simulink library "casper_library_accumulators"  (Simulink 7.2)
settings: Solver=ode45  SolverMode=SingleTasking  StartTime=0.0  StopTime=10.0  RelTol=1e-3
values from neighbouring files (symbols this model uses):
  blockCountBits = ceil(log2(numBlocks))    [address_gen_vacc_v2_mask.m]
  blockRowBits = 0    [address_gen_vacc_v2_mask.m]
  comp = compi    [bus_accumulator_init.m]    (also in bus_addsub_init.m = comp*2; bus_convert_init.m; bus_logical_init.m = comp*2; bus_maddsub_init.m = max([compa, compb, compc]))
libraries: xbsIndex_r4 x698, xbsReplacements_r4 x61, casper_library_misc x17, xps_library x9
(part 2 of 5)

== system casper_library_accumulators/simple_bram_vacc ==
  new_acc : Inport
  din : Inport  Port=2
  Adder : xbsIndex_r4/AddSub  mode=Addition  use_carryin=off  use_carryout=off  en=off  latency=2  precision=User Defined  arith_type="Signed  (2's comp)"  n_bits=n_bits  bin_pt=bin_pt  quantization=Truncate  overflow=Wrap  dbl_ovrd=off  use_behavioral_HDL=on  hw_selection=Fabric  pipelined=off  use_rpm=on  block_type=addsub
      settings: xl_area=[0, 0, 0, 0, 0, 0, 0]  block_version=10.1.3
  Constant : xbsIndex_r4/Constant  const=0  gui_display_data_type=Fixed-point  arith_type=Signed (2's comp)  n_bits=n_bits  bin_pt=bin_pt  preci_type=Single  exp_width=8  frac_width=24  explicit_period=on  period=1  equ=P=C  opselect=C  inp2=PCIN>>17  opr=+  inp1=P  carry=CIN  dbl_ovrd=off  block_type=constant
  Mux : xbsIndex_r4/Mux  inputs=2  en=off  latency=0  precision=Full  arith_type="Signed  (2's comp)"  n_bits=8  bin_pt=2  quantization=Truncate  overflow=Wrap  dbl_ovrd=off  block_type=mux
      settings: xl_area=[0, 0, 0, 0, 0, 0, 0]
  delay_bram : Subsystem  mask(delay_bram){DelayLen=vec_len - 2, bram_latency=2}
      mask prompts: DelayLen "Delay By:"; bram_latency "BRAM Latency"
      mask help: A delay block that uses BRAM for its storage.
      mask init:
      | if (DelayLen <= bram_latency)
      | 	error('delay value must be greater than BRAM Latency');
      | end
      | BitWidth = max(ceil(log2(DelayLen)), 2);
      mask Help: eval('xlWeb(''http://casper.berkeley.edu/wiki/Delay_bram'')')
  pulse_ext : Subsystem  mask(pulse_ext){pulse_len=vec_len}
      mask prompts: pulse_len "Length of Pulse"
      mask help:
      | Extends a boolean signal to be high for the specified number of clocks after
      | the last high input.
      mask init:
      | bits = ceil(log2(pulse_len+1));
      mask Help: eval('xlWeb(''http://casper.berkeley.edu/wiki/Pulse_ext'')')
  dout : Outport
  valid : Outport  Port=2
  wires:
  Constant/1 -> Mux/3
  Mux/1 -> Adder/2
  pulse_ext/1(out) -> Mux/1, valid/1
  din/1 -> Adder/1
  new_acc/1 -> pulse_ext/1(in)
  delay_bram/1(Out1) -> Mux/2, dout/1
  Adder/1 -> delay_bram/1(In1)

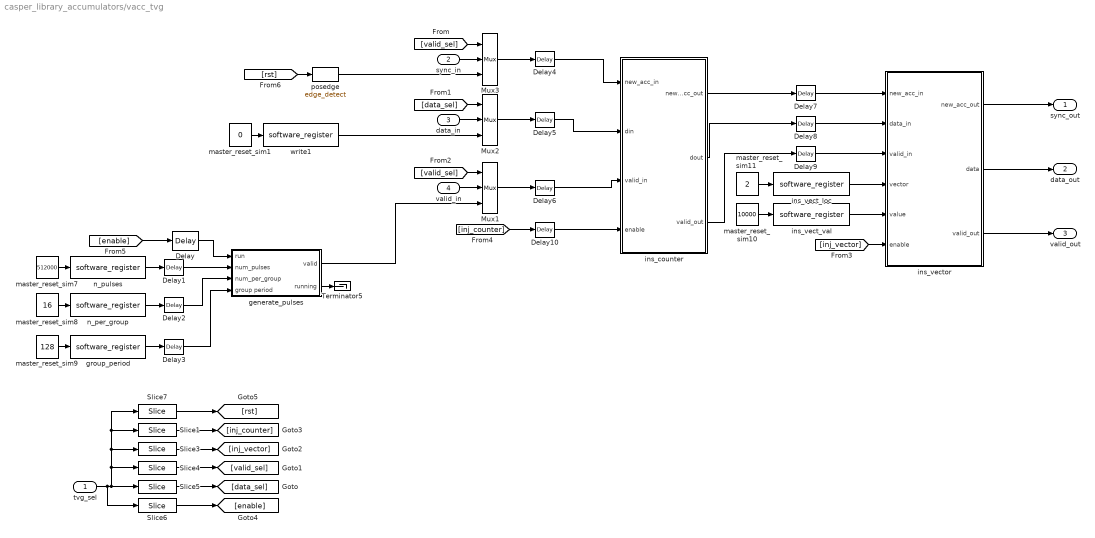
== system casper_library_accumulators/vacc_tvg ==
  tvg_sel : Inport
  sync_in : Inport  Port=2
  data_in : Inport  Port=3
  valid_in : Inport  Port=4
  Delay : xbsIndex_r4/Delay  rst=off  infoeditControl=Selection of Reset will increase slice count due to use of real FFs and instead of SRLs  en=off  latency=1  dbl_ovrd=off  reg_retiming=on  block_type=delay
      settings: xl_area=[0, 0, 0, 0, 0, 0, 0]
  Delay{1..10} (10 alike) : xbsIndex_r4/Delay  rst=off  infoeditControl=Selection of Reset will increase slice count due to use of real FFs and instead of SRLs  en=off  latency=2  dbl_ovrd=off  reg_retiming=on  block_type=delay
  Mux1 : xbsIndex_r4/Mux  inputs=2  en=off  latency=0  precision=Full  arith_type="Signed  (2's comp)"  n_bits=8  bin_pt=2  quantization=Truncate  overflow=Wrap  dbl_ovrd=off  block_type=mux
      settings: xl_area=[0, 0, 0, 0, 0, 0, 0]
  Mux2 : xbsIndex_r4/Mux  inputs=2  en=off  latency=0  precision=Full  arith_type="Signed  (2's comp)"  n_bits=8  bin_pt=2  quantization=Truncate  overflow=Wrap  dbl_ovrd=off  block_type=mux
      settings: xl_area=[0, 0, 0, 0, 0, 0, 0]
  Mux3 : xbsIndex_r4/Mux  inputs=2  en=off  latency=0  precision=Full  arith_type="Signed  (2's comp)"  n_bits=8  bin_pt=2  quantization=Truncate  overflow=Wrap  dbl_ovrd=off  block_type=mux
      settings: xl_area=[0, 0, 0, 0, 0, 0, 0]
  Slice1 : xbsIndex_r4/Slice  nbits=1  boolean_output=on  mode=Lower Bit Location + Width  bit1=0  base1=MSB of Input  bit0=4  base0=LSB of Input  dbl_ovrd=off  block_type=slice
      settings: infoedit="Extracts a given range of bits from each input sample and presents it at the output.  The output type is ordinarily unsigned with binary point at zero, but can be Boolean when the slice is one bit wide.<P><P>Hardware notes: In hardware this block costs nothing."  block_version=10.1.3
  Slice3 : xbsIndex_r4/Slice  nbits=1  boolean_output=on  mode=Lower Bit Location + Width  bit1=0  base1=MSB of Input  bit0=3  base0=LSB of Input  dbl_ovrd=off  block_type=slice
      settings: infoedit="Extracts a given range of bits from each input sample and presents it at the output.  The output type is ordinarily unsigned with binary point at zero, but can be Boolean when the slice is one bit wide.<P><P>Hardware notes: In hardware this block costs nothing."  block_version=10.1.3
  Slice4 : xbsIndex_r4/Slice  nbits=1  boolean_output=on  mode=Lower Bit Location + Width  bit1=0  base1=MSB of Input  bit0=2  base0=LSB of Input  dbl_ovrd=off  block_type=slice
      settings: infoedit="Extracts a given range of bits from each input sample and presents it at the output.  The output type is ordinarily unsigned with binary point at zero, but can be Boolean when the slice is one bit wide.<P><P>Hardware notes: In hardware this block costs nothing."  block_version=10.1.3
  Slice5 : xbsIndex_r4/Slice  nbits=1  boolean_output=on  mode=Lower Bit Location + Width  bit1=0  base1=MSB of Input  bit0=1  base0=LSB of Input  dbl_ovrd=off  block_type=slice
      settings: infoedit="Extracts a given range of bits from each input sample and presents it at the output.  The output type is ordinarily unsigned with binary point at zero, but can be Boolean when the slice is one bit wide.<P><P>Hardware notes: In hardware this block costs nothing."  block_version=10.1.3
  Slice6 : xbsIndex_r4/Slice  nbits=1  boolean_output=on  mode=Lower Bit Location + Width  bit1=0  base1=MSB of Input  bit0=0  base0=LSB of Input  dbl_ovrd=off  block_type=slice
      settings: infoedit="Extracts a given range of bits from each input sample and presents it at the output.  The output type is ordinarily unsigned with binary point at zero, but can be Boolean when the slice is one bit wide.<P><P>Hardware notes: In hardware this block costs nothing."  block_version=10.1.3
  Slice7 : xbsIndex_r4/Slice  nbits=1  boolean_output=on  mode=Lower Bit Location + Width  bit1=0  base1=MSB of Input  bit0=5  base0=LSB of Input  dbl_ovrd=off  block_type=slice
      settings: infoedit="Extracts a given range of bits from each input sample and presents it at the output.  The output type is ordinarily unsigned with binary point at zero, but can be Boolean when the slice is one bit wide.<P><P>Hardware notes: In hardware this block costs nothing."  block_version=10.1.3
  Terminator5 : Terminator
  generate_pulses : Subsystem
  group_period : xps_library/software_register  Tag=xps:sw_reg  SystemSampleTime=-1  io_dir=From Processor  arith_type=Unsigned  bitwidth=32  bin_pt=0  sample_period=1  gw_name=casper_library_accumulators_vacc_tvg_group_period_user_data_out
  ins_counter : Subsystem  mask{vec_len=len}
      mask prompts: vec_len "Vector Length?"
      mask init:
      | fmtstr = sprintf('Vector Length: %d', vec_len);
      | set_param(gcb, 'AttributesFormatString', fmtstr);
      settings: AttributesFormatString=Vector Length: 139264
  ins_vect_loc : xps_library/software_register  Tag=xps:sw_reg  SystemSampleTime=-1  io_dir=From Processor  arith_type=Unsigned  bitwidth=32  bin_pt=0  sample_period=1  gw_name=casper_library_accumulators_vacc_tvg_ins_vect_loc_user_data_out
  ins_vect_val : xps_library/software_register  Tag=xps:sw_reg  SystemSampleTime=-1  io_dir=From Processor  arith_type=Unsigned  bitwidth=32  bin_pt=0  sample_period=1  gw_name=casper_library_accumulators_vacc_tvg_ins_vect_val_user_data_out
  ins_vector : Subsystem  mask{num_vectors=len}
      mask prompts: num_vectors "number of vectors"
      mask init:
      | fmtstr = sprintf('Vector Length: %d', num_vectors);
      | set_param(gcb, 'AttributesFormatString', fmtstr);
      settings: AttributesFormatString=Vector Length: 139264
  master_reset_sim1 : Constant  Value=0
  master_reset_sim10 : Constant  Value=10000
  master_reset_sim11 : Constant  Value=2
  master_reset_sim7 : Constant  Value=512000
  master_reset_sim8 : Constant  Value=16
  master_reset_sim9 : Constant  Value=128
  n_per_group : xps_library/software_register  Tag=xps:sw_reg  SystemSampleTime=-1  io_dir=From Processor  arith_type=Unsigned  bitwidth=32  bin_pt=0  sample_period=1  gw_name=casper_library_accumulators_vacc_tvg_n_per_group_user_data_out
  n_pulses : xps_library/software_register  Tag=xps:sw_reg  SystemSampleTime=-1  io_dir=From Processor  arith_type=Unsigned  bitwidth=32  bin_pt=0  sample_period=1  gw_name=casper_library_accumulators_vacc_tvg_n_pulses_user_data_out
  posedge : casper_library_misc/edge_detect  SystemSampleTime=-1  edge=Rising  polarity=Active High  x_in=[0 0.08 0.08 0.16 0.16 0.24 0.24 0.32 0.32 0.4]  y_in="[-1 -1  1  1  1  1  1  1  1  1]"  x_out=[0.6 0.68 0.68 0.76 0.76 0.84 0.84 0.92 0.92 1]  y_out="[-1 -1  1  1 -1 -1 -1 -1 -1 -1]"
  write1 : xps_library/software_register  Tag=xps:sw_reg  SystemSampleTime=-1  io_dir=From Processor  arith_type=Unsigned  bitwidth=32  bin_pt=0  sample_period=1  gw_name=casper_library_accumulators_vacc_tvg_write1_user_data_out
  sync_out : Outport
  data_out : Outport  Port=2
  valid_out : Outport  Port=3
  wires:
  Delay10/1 -> ins_counter/4(enable)
  Delay9/1 -> ins_vector/3(valid_in)
  Delay8/1 -> ins_vector/2(data_in)
  Delay7/1 -> ins_vector/1(new_acc_in)
  Delay6/1 -> ins_counter/3(valid_in)
  Delay5/1 -> ins_counter/2(din)
  Delay4/1 -> ins_counter/1(new_acc_in)
  Delay3/1 -> generate_pulses/4(group period)
  Delay2/1 -> generate_pulses/3(num_per_group)
  Delay1/1 -> generate_pulses/2(num_pulses)
  write1/1 -> Mux2/3
  master_reset_sim1/1 -> write1/1
  [rst] -> posedge/1
  n_pulses/1 -> Delay1/1
  master_reset_sim7/1 -> n_pulses/1
  n_per_group/1 -> Delay2/1
  master_reset_sim8/1 -> n_per_group/1
  group_period/1 -> Delay3/1
  master_reset_sim9/1 -> group_period/1
  Mux1/1 -> Delay6/1
  valid_in/1 -> Mux1/2
  ins_vector/1(new_acc_out) -> sync_out/1
  ins_vector/2(data) -> data_out/1
  ins_vector/3(valid_out) -> valid_out/1
  ins_counter/1(new_acc_out) -> Delay7/1
  Mux2/1 -> Delay5/1
  data_in/1 -> Mux2/2
  sync_in/1 -> Mux3/2
  Mux3/1 -> Delay4/1
  Slice5/1 -> [data_sel]
  tvg_sel/1 -> Slice5/1, Slice3/1, Slice1/1, Slice7/1, Slice4/1, Slice6/1
  Slice4/1 -> [valid_sel]
  [valid_sel] -> Mux3/1
  [data_sel] -> Mux2/1
  [valid_sel] -> Mux1/1
  Slice3/1 -> [inj_vector]
  Slice1/1 -> [inj_counter]
  [enable] -> Delay/1
  ins_counter/2(dout) -> Delay8/1
  ins_counter/3(valid_out) -> Delay9/1
  generate_pulses/1(valid) -> Mux1/3
  posedge/1 -> Mux3/3
  [inj_vector] -> ins_vector/6(enable)
  master_reset_sim11/1 -> ins_vect_loc/1
  ins_vect_loc/1 -> ins_vector/4(vector)
  master_reset_sim10/1 -> ins_vect_val/1
  ins_vect_val/1 -> ins_vector/5(value)
  [inj_counter] -> Delay10/1
  Slice6/1 -> [enable]
  Slice7/1 -> [rst]
  Delay/1 -> generate_pulses/1(run)
  generate_pulses/2(running) -> Terminator5/1

== system casper_library_accumulators/wide_bram_vacc ==
  note: ALUMODE = 0 implements X+Y+Z+CIN
      | OPMODE selects X,Y,Z:
      | X is 0 (dv=0) or A:B (dv=1)
      | Y is 0 (acc=0) or C (acc=1)
      | Z is 0
      | CIN is CARRYIN (CARRYINSEL=0) (DSP48_low)
      | CIN is CARRYCASCIN (CARRYINSEL=2) (DSP48_high)
  new_acc : Inport
  din : Inport  Port=2
  dok : Inport  Port=3
  BitBasher : xbsIndex_r4/BitBasher  bitexpr=|  display_expr=off  sr_1=1  arith_type1="Signed  (2's comp)"  bin_pt1=0  sr_2=2  arith_type2="Signed  (2's comp)"  bin_pt2=0  sr_3=3  arith_type3=Unsigned  bin_pt3=0  sr_4=4  arith_type4=Unsigned  bin_pt4=0  dbl_ovrd=off  block_type=bitbasher
      | <!DOCTYPE HTML PUBLIC "-//W3C//DTD HTML 4.0//EN" "http://www.w3.org/TR/REC-html40/strict.dtd">
      | <html><head><meta name="qrichtext" content="1" /><style type="text/css">
      | p, li { white-space: pre-wrap; }
      | </style></head><body style=" font-family:'Sans'; font-size:10pt; font-weight:400; font-style:normal;">
      | <p style=" margin-top:12px; margin-bottom:12px; margin-left:0px; margin-right:0px; -qt-block-indent:0; text-indent:0px;"><span style=" font-family:'MS Shell Dlg'; font-size:8pt;">a={in[47:18]}<br />b={in[17:0]}</span></p></body></html>
  BitBasher1 : xbsIndex_r4/BitBasher  bitexpr=|  display_expr=off  sr_1=1  arith_type1=Unsigned  bin_pt1=0  sr_2=2  arith_type2=Unsigned  bin_pt2=0  sr_3=3  arith_type3=Unsigned  bin_pt3=0  sr_4=4  arith_type4=Unsigned  bin_pt4=0  dbl_ovrd=off  block_type=bitbasher
      | <!DOCTYPE HTML PUBLIC "-//W3C//DTD HTML 4.0//EN" "http://www.w3.org/TR/REC-html40/strict.dtd">
      | <html><head><meta name="qrichtext" content="1" /><style type="text/css">
      | p, li { white-space: pre-wrap; }
      | </style></head><body style=" font-family:'Sans'; font-size:10pt; font-weight:400; font-style:normal;">
      | <p style=" margin-top:12px; margin-bottom:12px; margin-left:0px; margin-right:0px; -qt-block-indent:0; text-indent:0px;"><span style=" font-family:'MS Shell Dlg'; font-size:8pt;">op={3'b000, acc, acc, dv, dv}</span></p></body></html>
  BitBasher3 : xbsIndex_r4/BitBasher  bitexpr=|  display_expr=off  sr_1=1  arith_type1="Signed  (2's comp)"  bin_pt1=0  sr_2=2  arith_type2="Signed  (2's comp)"  bin_pt2=0  sr_3=3  arith_type3=Unsigned  bin_pt3=0  sr_4=4  arith_type4=Unsigned  bin_pt4=0  dbl_ovrd=off  block_type=bitbasher
      | <!DOCTYPE HTML PUBLIC "-//W3C//DTD HTML 4.0//EN" "http://www.w3.org/TR/REC-html40/strict.dtd">
      | <html><head><meta name="qrichtext" content="1" /><style type="text/css">
      | p, li { white-space: pre-wrap; }
      | </style></head><body style=" font-family:'Sans'; font-size:10pt; font-weight:400; font-style:normal;">
      | <p style=" margin-top:12px; margin-bottom:12px; margin-left:0px; margin-right:0px; -qt-block-indent:0; text-indent:0px;"><span style=" font-family:'MS Shell Dlg'; font-size:8pt;">a={in[47:18]}<br />b={in[17:0]}</span></p></body></html>
  Constant10 : xbsIndex_r4/Constant  const=2  gui_display_data_type=Fixed-point  arith_type=Unsigned  n_bits=3  bin_pt=0  preci_type=Single  exp_width=8  frac_width=24  explicit_period=on  period=1  equ=P=C  opselect=C  inp2=PCIN>>17  opr=+  inp1=P  carry=CIN  dbl_ovrd=off  block_type=constant
  Constant11 : xbsIndex_r4/Constant  const=0  gui_display_data_type=Fixed-point  arith_type=Unsigned  n_bits=4  bin_pt=0  preci_type=Single  exp_width=8  frac_width=24  explicit_period=off  period=1  equ=P=C  opselect=C  inp2=PCIN>>17  opr=+  inp1=P  carry=CIN  dbl_ovrd=off  block_type=constant
  Constant12 : xbsIndex_r4/Constant  const=0  gui_display_data_type=Fixed-point  arith_type=Unsigned  n_bits=1  bin_pt=0  preci_type=Single  exp_width=8  frac_width=24  explicit_period=on  period=1  equ=P=C  opselect=C  inp2=PCIN>>17  opr=+  inp1=P  carry=CIN  dbl_ovrd=off  block_type=constant
  Constant13 : xbsIndex_r4/Constant  const=0  gui_display_data_type=Fixed-point  arith_type=Unsigned  n_bits=3  bin_pt=0  preci_type=Single  exp_width=8  frac_width=24  explicit_period=on  period=1  equ=P=C  opselect=C  inp2=PCIN>>17  opr=+  inp1=P  carry=CIN  dbl_ovrd=off  block_type=constant
  Constant8 : xbsIndex_r4/Constant  const=0  gui_display_data_type=Fixed-point  arith_type=Unsigned  n_bits=4  bin_pt=0  preci_type=Single  exp_width=8  frac_width=24  explicit_period=on  period=1  equ=P=C  opselect=C  inp2=PCIN>>17  opr=+  inp1=P  carry=CIN  dbl_ovrd=off  block_type=constant
  Constant9 : xbsIndex_r4/Constant  const=0  gui_display_data_type=Fixed-point  arith_type=Unsigned  n_bits=1  bin_pt=0  preci_type=Single  exp_width=8  frac_width=24  explicit_period=on  period=1  equ=P=C  opselect=C  inp2=PCIN>>17  opr=+  inp1=P  carry=CIN  dbl_ovrd=off  block_type=constant
  DSP48E1_high : xbsIndex_r4/DSP48E1   use_a=Direct from A Port  use_b=Direct from B Port  addsub_mode=ONE48  xl_useadderonly=on  xl_dynamicmult=off  enable_preadder=off  reset_preg=off  pattern_from_creg=1  pattern='000000000000'  mask_from_creg=1  pattern_mask='000000000000'  use_op=off  use_creg=on  rst_all=off  en_all=off  use_pcin=off  use_carrycascin=on  use_multsignin=off  use_carryout=off  use_patterndetect=off  use_patternbdetect=off  use_overflow=off  use_underflow=off  use_acout=off  use_bcout=off  use_pcout=off  use_multsignout=off  use_carrycascout=off  pipeline_a=2  pipeline_b=2  pipeline_acout=1  pipeline_bcout=1  pipeline_c=on  pipeline_p=on  pipeline_mult=off  pipeline_opmode=on  pipeline_alumode=off  pipeline_carryin=off  pipeline_carryinsel=off  dreg=off  adreg=off  register_inmode=off  rst_a=off  rst_b=off  rst_c=off  rst_mult=off  rst_p=off  rst_carry_in=off  rst_alumode=off  rst_ctrl=off  reset_port_d=off  reset_port_inmode=off  en_a1=off  en_a2=off  en_b1=off  en_b2=off  en_c=off  en_mult=off  en_p=off  en_carry_in=off  en_alumode=off  en_multcarryin=off  en_ctrl=off  enable_port_regd=off  enable_port_regad=off  enable_port_reginmode=off  use_synth_model=off  block_type=dsp48e1
  DSP48E1_low : xbsIndex_r4/DSP48E1   use_a=Direct from A Port  use_b=Direct from B Port  addsub_mode=ONE48  xl_useadderonly=on  xl_dynamicmult=off  enable_preadder=off  reset_preg=off  pattern_from_creg=1  pattern='000000000000'  mask_from_creg=1  pattern_mask='000000000000'  use_op=off  use_creg=on  rst_all=off  en_all=off  use_pcin=off  use_carrycascin=off  use_multsignin=off  use_carryout=off  use_patterndetect=off  use_patternbdetect=off  use_overflow=off  use_underflow=off  use_acout=off  use_bcout=off  use_pcout=off  use_multsignout=off  use_carrycascout=on  pipeline_a=1  pipeline_b=1  pipeline_acout=1  pipeline_bcout=1  pipeline_c=on  pipeline_p=on  pipeline_mult=off  pipeline_opmode=on  pipeline_alumode=off  pipeline_carryin=off  pipeline_carryinsel=off  dreg=off  adreg=off  register_inmode=off  rst_a=off  rst_b=off  rst_c=off  rst_mult=off  rst_p=off  rst_carry_in=off  rst_alumode=off  rst_ctrl=off  reset_port_d=off  reset_port_inmode=off  en_a1=off  en_a2=off  en_b1=off  en_b2=off  en_c=off  en_mult=off  en_p=off  en_carry_in=off  en_alumode=off  en_multcarryin=off  en_ctrl=off  enable_port_regd=off  enable_port_regad=off  enable_port_reginmode=off  use_synth_model=off  block_type=dsp48e1
  Delay : xbsIndex_r4/Delay  rst=off  infoeditControl=Selection of Reset will increase slice count due to use of real FFs and instead of SRLs  en=off  latency=1  dbl_ovrd=off  reg_retiming=on  block_type=delay
  Delay1 : xbsIndex_r4/Delay  rst=off  infoeditControl=Selection of Reset will increase slice count due to use of real FFs and instead of SRLs  en=off  latency=1  dbl_ovrd=off  reg_retiming=on  block_type=delay
  Delay2 : xbsIndex_r4/Delay  rst=off  infoeditControl=Selection of Reset will increase slice count due to use of real FFs and instead of SRLs  en=off  latency=1  dbl_ovrd=off  reg_retiming=on  block_type=delay
  Inverter : xbsIndex_r4/Inverter  en=off  latency=0  dbl_ovrd=off  block_type=inv
  delay_bram_high : Subsystem  mask(delay_bram){DelayLen=vec_len - 2, bram_latency=2}
      mask prompts: DelayLen "Delay By:"; bram_latency "BRAM Latency"
      mask help: A delay block that uses BRAM for its storage.
      mask init:
      | if (DelayLen <= bram_latency)
      | 	error('delay value must be greater than BRAM Latency');
      | end
      | BitWidth = max(ceil(log2(DelayLen)), 2);
      mask Help: eval('xlWeb(''http://casper.berkeley.edu/wiki/Delay_bram'')')
  delay_bram_low : Subsystem  mask(delay_bram){DelayLen=vec_len - 2, bram_latency=2}
      mask prompts: DelayLen "Delay By:"; bram_latency "BRAM Latency"
      mask help: A delay block that uses BRAM for its storage.
      mask init:
      | if (DelayLen <= bram_latency)
      | 	error('delay value must be greater than BRAM Latency');
      | end
      | BitWidth = max(ceil(log2(DelayLen)), 2);
      mask Help: eval('xlWeb(''http://casper.berkeley.edu/wiki/Delay_bram'')')
  insize : Subsystem
  outsize : Subsystem
  pulse_ext : Subsystem  mask(pulse_ext){pulse_len=vec_len}
      mask prompts: pulse_len "Length of Pulse"
      mask help:
      | Extends a boolean signal to be high for the specified number of clocks after
      | the last high input.
      mask init:
      | bits = ceil(log2(pulse_len+1));
      mask Help: eval('xlWeb(''http://casper.berkeley.edu/wiki/Pulse_ext'')')
  dout : Outport
  valid : Outport  Port=2
  wires:
  new_acc/1 -> pulse_ext/1(in)  "new_acc"
  pulse_ext/1(out) -> Inverter/1, Delay2/1  "init"
  DSP48E1_low/2 -> DSP48E1_high/8  "carry"
  BitBasher/1 -> DSP48E1_low/1  "lo_a"
  BitBasher/2 -> DSP48E1_low/2  "lo_b"
  DSP48E1_low/1 -> delay_bram_low/1(In1)  "lo_p"
  delay_bram_low/1(Out1) -> Delay/1, DSP48E1_low/3  "lo_c"
  BitBasher1/1 -> Delay1/1, DSP48E1_low/4  "lo_op"
  Inverter/1 -> BitBasher1/1  "acc"
  dok/1 -> BitBasher1/2  "dok"
  BitBasher3/1 -> DSP48E1_high/1  "hi_a"
  BitBasher3/2 -> DSP48E1_high/2  "hi_b"
  Delay1/1 -> DSP48E1_high/4  "hi_op"
  Constant8/1 -> DSP48E1_high/5
  Constant9/1 -> DSP48E1_high/6
  Constant10/1 -> DSP48E1_high/7
  DSP48E1_high/1 -> delay_bram_high/1(In1)  "hi_p"
  Constant11/1 -> DSP48E1_low/5
  Constant12/1 -> DSP48E1_low/6
  Constant13/1 -> DSP48E1_low/7
  din/1 -> insize/1(in)  "din"
  insize/2(lo) -> BitBasher/1  "lo"
  delay_bram_high/1(Out1) -> outsize/1(hi), DSP48E1_high/3  "hi_c"
  insize/1(hi) -> BitBasher3/1  "hi"
  Delay/1 -> outsize/2(lo)  "lo_c1"
  outsize/1(out) -> dout/1  "dout"
  Delay2/1 -> valid/1  "valid"

== system casper_library_accumulators/addr_bram_vacc/delay_bram ==
  In1 : Inport
  Constant2 : xbsIndex_r4/Constant  const=1  gui_display_data_type=Fixed-point  arith_type=Boolean  n_bits=1  bin_pt=0  preci_type=Single  exp_width=8  frac_width=24  explicit_period=on  period=1  equ=P=C  opselect=C  inp2=PCIN>>17  opr=+  inp1=P  carry=CIN  dbl_ovrd=off  block_type=constant
  Counter : xbsIndex_r4/Counter  cnt_type=Count Limited  cnt_to=DelayLen - bram_latency - 1  operation=Up  start_count=0  cnt_by_val=1  arith_type=Unsigned  n_bits=BitWidth  bin_pt=0  load_pin=off  rst=off  en=off  explicit_period=off  period=1  dbl_ovrd=off  use_behavioral_HDL=on  implementation=Fabric  use_rpm=off  block_type=counter
      settings: xl_area=[0, 0, 0, 0, 0, 0, 0]
  Single Port RAM : xbsIndex_r4/Single Port RAM  depth=2^BitWidth  initVector=0  distributed_mem=Block RAM  write_mode=Read Before Write  rst=off  init_reg=0  en=off  latency=bram_latency  dbl_ovrd=off  optimize=Area  use_rpm=off  block_type=spram
      settings: xl_area=[0, 0, 0, 0, 0, 0, 0]  block_version=10.1.3
  Out1 : Outport
  wires:
  Single Port RAM/1 -> Out1/1
  Counter/1 -> Single Port RAM/1
  In1/1 -> Single Port RAM/2
  Constant2/1 -> Single Port RAM/3

== system casper_library_accumulators/addr_bram_vacc/pulse_ext ==
  in : Inport
  Constant5 : xbsIndex_r4/Constant  const=pulse_len  gui_display_data_type=Fixed-point  arith_type=Unsigned  n_bits=bits  bin_pt=0  preci_type=Single  exp_width=8  frac_width=24  explicit_period=off  period=1  equ=P=C  opselect=C  inp2=PCIN>>17  opr=+  inp1=P  carry=CIN  dbl_ovrd=off  block_type=constant
  Counter3 : xbsIndex_r4/Counter  cnt_type=Free Running  cnt_to=1023  operation=Up  start_count=0  cnt_by_val=1  arith_type=Unsigned  n_bits=bits  bin_pt=0  load_pin=off  rst=on  en=on  explicit_period=on  period=1  dbl_ovrd=off  use_behavioral_HDL=on  implementation=Fabric  use_rpm=on  block_type=counter
      settings: xl_area=[0, 0, 0, 0, 0, 0, 0]
  Relational5 : xbsIndex_r4/Relational  mode=a!=b  en=off  latency=0  dbl_ovrd=off  block_type=relational
      settings: xl_area=[0, 0, 0, 0, 0, 0, 0]  block_version=10.1.3
  posedge : Subsystem  Tag=Rising Edge Detector
  out : Outport
  wires:
  posedge/1(Out) -> Counter3/1
  in/1 -> posedge/1(In)
  Relational5/1 -> out/1, Counter3/2
  Constant5/1 -> Relational5/2
  Counter3/1 -> Relational5/1

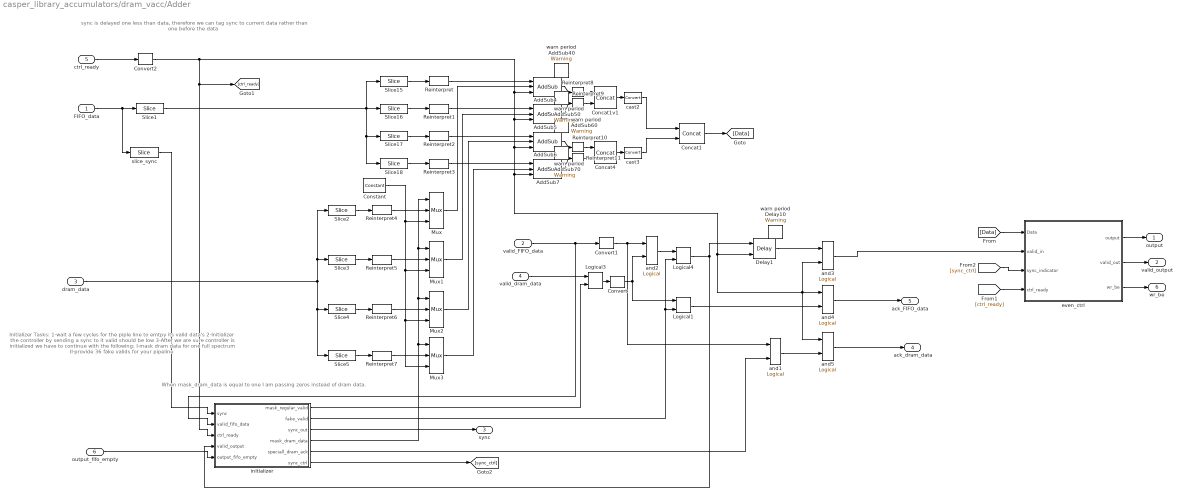
== system casper_library_accumulators/dram_vacc/Adder ==
  note: When mask_dram_data is equal to one
      | I am passing zeros instead of dram data.
  note: Initializer Tasks:
      | 1-wait a few cycles for the piple line to emtpy
      | its valid data's
      | 2-Initializer the controller by sending a sync to it
      | valid should be low
      | 3-After we are sure controller is initialized we have to
      | continue with the following:
      | I-mask dram data for one full spectrum
      | II-provide 36 fake valids for your pipeline
  note: sync is delayed one less than data,
      | therefore we can tag sync to current data rather than
      | one before the data
  FIFO_data : Inport
  valid_FIFO_data : Inport  Port=2
  dram_data : Inport  Port=3
  valid_dram_data : Inport  Port=4
  ctrl_ready : Inport  Port=5
  output_fifo_empty : Inport  Port=6
  AddSub{4..7} (4 alike) : xbsIndex_r4/AddSub  mode=Addition  use_carryin=off  use_carryout=off  en=on  latency=3  precision=User Defined  arith_type="Signed  (2's comp)"  n_bits=32  bin_pt=0  quantization="Round  (unbiased: +/- Inf)"  overflow=Wrap  dbl_ovrd=off  use_behavioral_HDL=on  hw_selection=Fabric  pipelined=on  use_rpm=on  block_type=addsub
      settings: xl_area=[0, 0, 0, 0, 0, 0, 0]  block_version=9.2.01
  Concat1 : xbsIndex_r4/Concat  num_inputs=2  dbl_ovrd=off  block_type=concat
      settings: block_version=9.2.01
  Concat1v1 : xbsIndex_r4/Concat  num_inputs=2  dbl_ovrd=off  block_type=concat
      settings: block_version=9.2.01
  Concat4 : xbsIndex_r4/Concat  num_inputs=2  dbl_ovrd=off  block_type=concat
      settings: block_version=9.2.01
  Constant : xbsIndex_r4/Constant  const=0  gui_display_data_type=Fixed-point  arith_type=Signed (2's comp)  n_bits=32  bin_pt=0  preci_type=Single  exp_width=8  frac_width=24  explicit_period=on  period=1  equ=P=C  opselect=C  inp2=PCIN>>17  opr=+  inp1=P  carry=CIN  dbl_ovrd=off  block_type=constant
      settings: block_version=9.2.01
  Convert : xbsIndex_r4/Convert  gui_display_data_type=Fixed-point  arith_type=Boolean  n_bits=8  bin_pt=6  float_type=Single  exp_bits=8  fraction_bits=24  quantization=Truncate  overflow=Wrap  en=off  latency=0  dbl_ovrd=off  pipeline=off  block_type=convert
      settings: xl_area=[0, 0, 0, 0, 0, 0, 0]  block_version=9.2.01
  Convert1 : xbsIndex_r4/Convert  gui_display_data_type=Fixed-point  arith_type=Boolean  n_bits=8  bin_pt=6  float_type=Single  exp_bits=8  fraction_bits=24  quantization=Truncate  overflow=Wrap  en=off  latency=0  dbl_ovrd=off  pipeline=off  block_type=convert
      settings: xl_area=[0, 0, 0, 0, 0, 0, 0]  block_version=9.2.01
  Convert2 : xbsIndex_r4/Convert  gui_display_data_type=Fixed-point  arith_type=Boolean  n_bits=8  bin_pt=6  float_type=Single  exp_bits=8  fraction_bits=24  quantization=Truncate  overflow=Wrap  en=off  latency=0  dbl_ovrd=off  pipeline=off  block_type=convert
      settings: xl_area=[0, 0, 0, 0, 0, 0, 0]  block_version=9.2.01
  Delay1 : xbsIndex_r4/Delay  rst=off  infoeditControl=Selection of Reset will increase slice count due to use of real FFs and instead of SRLs  en=on  latency=3  dbl_ovrd=off  reg_retiming=on  block_type=delay
      settings: xl_area=[0, 0, 0, 0, 0, 0, 0]  block_version=9.2.01
  Logical1 : xbsIndex_r4/Logical  logical_function=OR  inputs=2  en=off  latency=0  precision=Full  arith_type=Unsigned  n_bits=8  bin_pt=2  align_bp=on  dbl_ovrd=off  block_type=logical
      settings: xl_area=[0, 0, 0, 0, 0, 0, 0]  block_version=9.2.01
  Logical3 : xbsIndex_r4/Logical  logical_function=AND  inputs=2  en=off  latency=0  precision=Full  arith_type=Unsigned  n_bits=8  bin_pt=2  align_bp=on  dbl_ovrd=off  block_type=logical
      settings: xl_area=[0, 0, 0, 0, 0, 0, 0]  block_version=9.2.01
  Logical4 : xbsIndex_r4/Logical  logical_function=OR  inputs=2  en=off  latency=0  precision=Full  arith_type=Unsigned  n_bits=8  bin_pt=2  align_bp=on  dbl_ovrd=off  block_type=logical
      settings: xl_area=[0, 0, 0, 0, 0, 0, 0]  block_version=9.2.01
  Mux{,1..3} (4 alike) : xbsIndex_r4/Mux  inputs=2  en=off  latency=0  precision=Full  arith_type="Signed  (2's comp)"  n_bits=8  bin_pt=2  quantization=Truncate  overflow=Wrap  dbl_ovrd=off  block_type=mux
      settings: xl_area=[0, 0, 0, 0, 0, 0, 0]  block_version=9.2.01
  Reinterpret{,1..7} (8 alike) : xbsIndex_r4/Reinterpret  force_arith_type=on  arith_type="Signed  (2's comp)"  force_bin_pt=on  bin_pt=0  block_type=reinterpret
      settings: infoedit="Changes signal type without altering the binary representation.   You can changed the signal between signed and unsigned, and relocate the binary point.<P><P>Hardware notes: In hardware this block costs nothing.<P><P>Example:  Suppose the input is 6 bits wide, signed, with 2 fractional bits, and the output is forced to unsigned with 0 fractional bits.  Then an input of -2.0 (1110.00 in binary 2's complement) becomes an output of 56 (111000 in binary)."  block_version=9.2.01
  Reinterpret{8..11} (4 alike) : xbsIndex_r4/Reinterpret  force_arith_type=on  arith_type=Unsigned  force_bin_pt=on  bin_pt=0  block_type=reinterpret
      settings: infoedit="Changes signal type without altering the binary representation.   You can changed the signal between signed and unsigned, and relocate the binary point.<P><P>Hardware notes: In hardware this block costs nothing.<P><P>Example:  Suppose the input is 6 bits wide, signed, with 2 fractional bits, and the output is forced to unsigned with 0 fractional bits.  Then an input of -2.0 (1110.00 in binary 2's complement) becomes an output of 56 (111000 in binary)."  block_version=9.2.01
  Slice1 : xbsIndex_r4/Slice  nbits=128  boolean_output=off  mode=Lower Bit Location + Width  bit1=0  base1=MSB of Input  bit0=0  base0=LSB of Input  dbl_ovrd=off  block_type=slice
      settings: infoedit="Extracts a given range of bits from each input sample and presents it at the output.  The output type is ordinarily unsigned with binary point at zero, but can be Boolean when the slice is one bit wide.<P><P>Hardware notes: In hardware this block costs nothing."  block_version=9.2.01
  Slice15 : xbsIndex_r4/Slice  nbits=32  boolean_output=off  mode=Lower Bit Location + Width  bit1=96  base1=MSB of Input  bit0=96  base0=LSB of Input  dbl_ovrd=off  block_type=slice
      settings: infoedit="Extracts a given range of bits from each input sample and presents it at the output.  The output type is ordinarily unsigned with binary point at zero, but can be Boolean when the slice is one bit wide.<P><P>Hardware notes: In hardware this block costs nothing."  block_version=9.2.01
  Slice16 : xbsIndex_r4/Slice  nbits=32  boolean_output=off  mode=Lower Bit Location + Width  bit1=-32  base1=MSB of Input  bit0=64  base0=LSB of Input  dbl_ovrd=off  block_type=slice
      settings: infoedit="Extracts a given range of bits from each input sample and presents it at the output.  The output type is ordinarily unsigned with binary point at zero, but can be Boolean when the slice is one bit wide.<P><P>Hardware notes: In hardware this block costs nothing."  block_version=9.2.01
  Slice17 : xbsIndex_r4/Slice  nbits=32  boolean_output=off  mode=Lower Bit Location + Width  bit1=0  base1=MSB of Input  bit0=32  base0=LSB of Input  dbl_ovrd=off  block_type=slice
      settings: infoedit="Extracts a given range of bits from each input sample and presents it at the output.  The output type is ordinarily unsigned with binary point at zero, but can be Boolean when the slice is one bit wide.<P><P>Hardware notes: In hardware this block costs nothing."  block_version=9.2.01
  Slice18 : xbsIndex_r4/Slice  nbits=32  boolean_output=off  mode=Lower Bit Location + Width  bit1=0  base1=MSB of Input  bit0=0  base0=LSB of Input  dbl_ovrd=off  block_type=slice
      settings: infoedit="Extracts a given range of bits from each input sample and presents it at the output.  The output type is ordinarily unsigned with binary point at zero, but can be Boolean when the slice is one bit wide.<P><P>Hardware notes: In hardware this block costs nothing."  block_version=9.2.01
  Slice2 : xbsIndex_r4/Slice  nbits=32  boolean_output=off  mode=Lower Bit Location + Width  bit1=0  base1=MSB of Input  bit0=104  base0=LSB of Input  dbl_ovrd=off  block_type=slice
      settings: infoedit="Extracts a given range of bits from each input sample and presents it at the output.  The output type is ordinarily unsigned with binary point at zero, but can be Boolean when the slice is one bit wide.<P><P>Hardware notes: In hardware this block costs nothing."  block_version=9.2.01
  Slice3 : xbsIndex_r4/Slice  nbits=32  boolean_output=off  mode=Lower Bit Location + Width  bit1=72  base1=MSB of Input  bit0=72  base0=LSB of Input  dbl_ovrd=off  block_type=slice
      settings: infoedit="Extracts a given range of bits from each input sample and presents it at the output.  The output type is ordinarily unsigned with binary point at zero, but can be Boolean when the slice is one bit wide.<P><P>Hardware notes: In hardware this block costs nothing."  block_version=9.2.01
  Slice4 : xbsIndex_r4/Slice  nbits=32  boolean_output=off  mode=Lower Bit Location + Width  bit1=0  base1=MSB of Input  bit0=32  base0=LSB of Input  dbl_ovrd=off  block_type=slice
      settings: infoedit="Extracts a given range of bits from each input sample and presents it at the output.  The output type is ordinarily unsigned with binary point at zero, but can be Boolean when the slice is one bit wide.<P><P>Hardware notes: In hardware this block costs nothing."  block_version=9.2.01
  Slice5 : xbsIndex_r4/Slice  nbits=32  boolean_output=off  mode=Lower Bit Location + Width  bit1=0  base1=MSB of Input  bit0=0  base0=LSB of Input  dbl_ovrd=off  block_type=slice
      settings: infoedit="Extracts a given range of bits from each input sample and presents it at the output.  The output type is ordinarily unsigned with binary point at zero, but can be Boolean when the slice is one bit wide.<P><P>Hardware notes: In hardware this block costs nothing."  block_version=9.2.01
  and1 : xbsIndex_r4/Logical  logical_function=OR  inputs=2  en=off  latency=0  precision=Full  arith_type=Unsigned  n_bits=8  bin_pt=2  align_bp=on  dbl_ovrd=off  block_type=logical
      settings: xl_area=[0, 0, 0, 0, 0, 0, 0]  block_version=9.2.01
  and{2..5} (4 alike) : xbsIndex_r4/Logical  logical_function=AND  inputs=2  en=off  latency=0  precision=Full  arith_type=Unsigned  n_bits=8  bin_pt=2  align_bp=on  dbl_ovrd=off  block_type=logical
      settings: xl_area=[0, 0, 0, 0, 0, 0, 0]  block_version=9.2.01
  cast2 : xbsIndex_r4/Convert  gui_display_data_type=Fixed-point  arith_type=Unsigned  n_bits=72  bin_pt=0  float_type=Single  exp_bits=8  fraction_bits=24  quantization=Truncate  overflow=Wrap  en=off  latency=0  dbl_ovrd=off  pipeline=off  block_type=convert
      settings: xl_area=[0, 0, 0, 0, 0, 0, 0]  block_version=9.2.01
  cast3 : xbsIndex_r4/Convert  gui_display_data_type=Fixed-point  arith_type=Unsigned  n_bits=72  bin_pt=0  float_type=Single  exp_bits=8  fraction_bits=24  quantization=Truncate  overflow=Wrap  en=off  latency=0  dbl_ovrd=off  pipeline=off  block_type=convert
      settings: xl_area=[0, 0, 0, 0, 0, 0, 0]  block_version=9.2.01
  even_ctrl : Subsystem
  initializer : Subsystem
  slice_sync : xbsIndex_r4/Slice  nbits=1  boolean_output=on  mode=Upper Bit Location + Width  bit1=0  base1=MSB of Input  bit0=0  base0=LSB of Input  dbl_ovrd=off  block_type=slice
      settings: infoedit="Extracts a given range of bits from each input sample and presents it at the output.  The output type is ordinarily unsigned with binary point at zero, but can be Boolean when the slice is one bit wide.<P><P>Hardware notes: In hardware this block costs nothing."  block_version=9.2.01
  warn period AddSub{40,50,60,70} (4 alike) : xbsReplacements_r4/Warning  SystemSampleTime=-1  period=1
  warn period Delay10 : xbsReplacements_r4/Warning  SystemSampleTime=-1  period=1
  output : Outport
  valid_output : Outport  Port=2
  sync : Outport  Port=3
  ack_dram_data : Outport  Port=4
  ack_FIFO_data : Outport  Port=5
  wr_be : Outport  Port=6
  wires:
  Reinterpret11/1 -> Concat4/2
  Reinterpret10/1 -> Concat4/1
  Reinterpret9/1 -> Concat1v1/2
  Reinterpret8/1 -> Concat1v1/1
  Reinterpret7/1 -> Mux3/2
  Reinterpret6/1 -> Mux2/2
  Reinterpret5/1 -> Mux1/2
  Reinterpret4/1 -> Mux/2
  Reinterpret3/1 -> AddSub7/1
  Reinterpret2/1 -> AddSub6/1
  Reinterpret1/1 -> AddSub5/1
  Reinterpret/1 -> AddSub4/1
  Logical1/1 -> and4/2
  and1/1 -> and5/2
  and5/1 -> ack_dram_data/1
  Logical4/1 -> initializer/4(valid_output), Delay1/1
  initializer/5(speciall_dram_ack) -> and1/2
  output_fifo_empty/1 -> initializer/5(output_fifo_empty)
  Constant/1 -> Mux2/3, Mux3/3, Mux1/3, Mux/3
  initializer/4(mask_dram_data) -> Mux3/1, Mux2/1, Mux1/1, Mux/1
  Slice2/1 -> Reinterpret4/1
  Slice3/1 -> Reinterpret5/1
  Slice4/1 -> Reinterpret6/1
  Slice5/1 -> Reinterpret7/1
  initializer/3(sync_out) -> sync/1
  and2/1 -> Logical4/1
  and4/1 -> ack_FIFO_data/1
  Delay1/1 -> and3/1
  initializer/2(fake_valid) -> Logical1/2, Logical4/2
  Logical3/1 -> Convert/1
  initializer/1(mask_regular_valid) -> Logical3/2
  valid_dram_data/1 -> Logical3/1
  and3/1 -> even_ctrl/2(valid_in)
  Convert2/1 -> [ctrl_ready], initializer/3(ctrl_ready), AddSub4/3, AddSub5/3, Delay1/2, and5/1, and4/1, and3/2, AddSub7/3, AddSub6/3
  Convert1/1 -> and1/1, and2/1
  Convert/1 -> Logical1/1, and2/2
  slice_sync/1 -> initializer/1(sync)
  Slice1/1 -> Slice18/1, Slice17/1, Slice16/1, Slice15/1
  dram_data/1 -> Slice4/1, Slice5/1, Slice3/1, Slice2/1
  valid_FIFO_data/1 -> Convert1/1, initializer/2(valid_fifo_data)
  ctrl_ready/1 -> Convert2/1
  FIFO_data/1 -> slice_sync/1, Slice1/1
  cast3/1 -> Concat1/2
  Concat4/1 -> cast3/1
  cast2/1 -> Concat1/1
  Concat1v1/1 -> cast2/1
  AddSub7/1 -> Reinterpret11/1
  AddSub6/1 -> Reinterpret10/1
  AddSub5/1 -> Reinterpret9/1
  AddSub4/1 -> Reinterpret8/1
  Mux3/1 -> AddSub7/2
  Mux2/1 -> AddSub6/2
  Mux1/1 -> AddSub5/2
  Mux/1 -> AddSub4/2
  Slice18/1 -> Reinterpret3/1
  Slice17/1 -> Reinterpret2/1
  Slice16/1 -> Reinterpret1/1
  Slice15/1 -> Reinterpret/1
  even_ctrl/1(output) -> output/1
  even_ctrl/2(valid_out) -> valid_output/1
  Concat1/1 -> [Data]
  [Data] -> even_ctrl/1(Data)
  [ctrl_ready] -> even_ctrl/4(ctrl_ready)
  even_ctrl/3(wr_be) -> wr_be/1
  initializer/6(sync_ctrl) -> [sync_ctrl]
  [sync_ctrl] -> even_ctrl/3(sync_indicator)

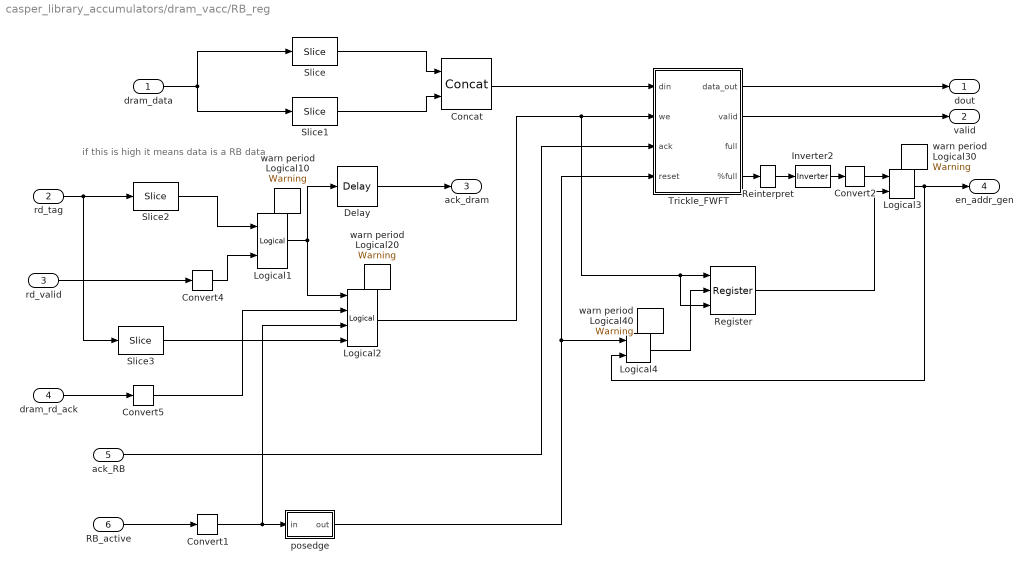
== system casper_library_accumulators/dram_vacc/RB_reg ==
  note: if this is high it means data is a RB data
  dram_data : Inport
  rd_tag : Inport  Port=2
  rd_valid : Inport  Port=3
  dram_rd_ack : Inport  Port=4
  ack_RB : Inport  Port=5
  RB_active : Inport  Port=6
  Concat : xbsIndex_r4/Concat  num_inputs=2  dbl_ovrd=off  block_type=concat
      settings: block_version=9.2.01
  Convert{1..2,4..5} (4 alike) : xbsIndex_r4/Convert  gui_display_data_type=Fixed-point  arith_type=Boolean  n_bits=31  bin_pt=0  float_type=Single  exp_bits=8  fraction_bits=24  quantization=Truncate  overflow=Wrap  en=off  latency=0  dbl_ovrd=off  pipeline=off  block_type=convert
      settings: xl_area=[0, 0, 0, 0, 0, 0, 0]  block_version=9.2.01
  Delay : xbsIndex_r4/Delay  rst=off  infoeditControl=Selection of Reset will increase slice count due to use of real FFs and instead of SRLs  en=off  latency=1  dbl_ovrd=off  reg_retiming=on  block_type=delay
      settings: xl_area=[0, 0, 0, 0, 0, 0, 0]  block_version=9.2.01
  Inverter2 : xbsIndex_r4/Inverter  en=off  latency=0  dbl_ovrd=off  block_type=inv
      settings: xl_area=[0, 0, 0, 0, 0, 0, 0]  block_version=9.2.01
  Logical1 : xbsIndex_r4/Logical  logical_function=AND  inputs=2  en=off  latency=0  precision=Full  arith_type=Unsigned  n_bits=8  bin_pt=2  align_bp=on  dbl_ovrd=off  block_type=logical
      settings: xl_area=[0, 0, 0, 0, 0, 0, 0]  block_version=9.2.01
  Logical2 : xbsIndex_r4/Logical  logical_function=AND  inputs=4  en=off  latency=0  precision=Full  arith_type=Unsigned  n_bits=8  bin_pt=2  align_bp=on  dbl_ovrd=off  block_type=logical
      settings: xl_area=[0, 0, 0, 0, 0, 0, 0]  block_version=9.2.01
  Logical3 : xbsIndex_r4/Logical  logical_function=AND  inputs=2  en=off  latency=0  precision=Full  arith_type=Unsigned  n_bits=8  bin_pt=2  align_bp=on  dbl_ovrd=off  block_type=logical
      settings: xl_area=[0, 0, 0, 0, 0, 0, 0]  block_version=9.2.01
  Logical4 : xbsIndex_r4/Logical  logical_function=OR  inputs=2  en=off  latency=0  precision=Full  arith_type=Unsigned  n_bits=8  bin_pt=2  align_bp=on  dbl_ovrd=off  block_type=logical
      settings: xl_area=[0, 0, 0, 0, 0, 0, 0]  block_version=9.2.01
  Register : xbsIndex_r4/Register  init=0  rst=on  en=on  dbl_ovrd=off  block_type=register
      settings: xl_area=[0, 0, 0, 0, 0, 0, 0]  block_version=9.2.01
  Reinterpret : xbsIndex_r4/Reinterpret  force_arith_type=on  arith_type=Unsigned  force_bin_pt=on  bin_pt=0  block_type=reinterpret
      settings: infoedit="Changes signal type without altering the binary representation.   You can changed the signal between signed and unsigned, and relocate the binary point.<P><P>Hardware notes: In hardware this block costs nothing.<P><P>Example:  Suppose the input is 6 bits wide, signed, with 2 fractional bits, and the output is forced to unsigned with 0 fractional bits.  Then an input of -2.0 (1110.00 in binary 2's complement) becomes an output of 56 (111000 in binary)."  block_version=9.2.01
  Slice : xbsIndex_r4/Slice  nbits=64  boolean_output=off  mode=Lower Bit Location + Width  bit1=0  base1=MSB of Input  bit0=72  base0=LSB of Input  dbl_ovrd=off  block_type=slice
      settings: infoedit="Extracts a given range of bits from each input sample and presents it at the output.  The output type is ordinarily unsigned with binary point at zero, but can be Boolean when the slice is one bit wide.<P><P>Hardware notes: In hardware this block costs nothing."  block_version=9.2.01
  Slice1 : xbsIndex_r4/Slice  nbits=64  boolean_output=off  mode=Lower Bit Location + Width  bit1=0  base1=MSB of Input  bit0=0  base0=LSB of Input  dbl_ovrd=off  block_type=slice
      settings: infoedit="Extracts a given range of bits from each input sample and presents it at the output.  The output type is ordinarily unsigned with binary point at zero, but can be Boolean when the slice is one bit wide.<P><P>Hardware notes: In hardware this block costs nothing."  block_version=9.2.01
  Slice2 : xbsIndex_r4/Slice  nbits=1  boolean_output=on  mode=Upper Bit Location + Width  bit1=0  base1=MSB of Input  bit0=74  base0=LSB of Input  dbl_ovrd=off  block_type=slice
      settings: infoedit="Extracts a given range of bits from each input sample and presents it at the output.  The output type is ordinarily unsigned with binary point at zero, but can be Boolean when the slice is one bit wide.<P><P>Hardware notes: In hardware this block costs nothing."  block_version=9.2.01
  Slice3 : xbsIndex_r4/Slice  nbits=1  boolean_output=on  mode=Lower Bit Location + Width  bit1=0  base1=MSB of Input  bit0=0  base0=LSB of Input  dbl_ovrd=off  block_type=slice
      settings: infoedit="Extracts a given range of bits from each input sample and presents it at the output.  The output type is ordinarily unsigned with binary point at zero, but can be Boolean when the slice is one bit wide.<P><P>Hardware notes: In hardware this block costs nothing."  block_version=9.2.01
  Trickle_FWFT : Subsystem  mask{depth=16}
      mask init:
      | cursys = gcb ; 
      | set_param([cursys, '/FIFO'], 'depth', depth);
      mask StyleString: popup(16|32|64|128|256|512|1K|2K|4K|8K|16K|32K|64K)
  posedge : Subsystem
  warn period Logical{10,20,30,40} (4 alike) : xbsReplacements_r4/Warning  SystemSampleTime=-1  period=1
  dout : Outport
  valid : Outport  Port=2
  ack_dram : Outport  Port=3
  en_addr_gen : Outport  Port=4
  wires:
  Reinterpret/1 -> Inverter2/1
  Convert2/1 -> Logical3/1
  Slice3/1 -> Logical2/4
  Slice2/1 -> Logical1/1
  Convert4/1 -> Logical1/2
  Logical4/1 -> Register/2
  Register/1 -> Logical3/2
  Logical3/1 -> Logical4/2, en_addr_gen/1
  Inverter2/1 -> Convert2/1
  Trickle_FWFT/4(%full) -> Reinterpret/1
  Trickle_FWFT/2(valid) -> valid/1
  Trickle_FWFT/1(data_out) -> dout/1
  posedge/1(out) -> Logical4/1, Trickle_FWFT/4(reset)
  Concat/1 -> Trickle_FWFT/1(din)
  ack_RB/1 -> Trickle_FWFT/3(ack)
  Convert1/1 -> Logical2/3, posedge/1(in)
  dram_data/1 -> Slice1/1, Slice/1
  Slice1/1 -> Concat/2
  Slice/1 -> Concat/1
  Convert5/1 -> Logical2/2
  RB_active/1 -> Convert1/1
  Logical2/1 -> Register/3, Register/1, Trickle_FWFT/2(we)
  dram_rd_ack/1 -> Convert5/1
  Logical1/1 -> Logical2/1, Delay/1
  Delay/1 -> ack_dram/1
  rd_valid/1 -> Convert4/1
  rd_tag/1 -> Slice3/1, Slice2/1

== system casper_library_accumulators/dram_vacc/Trickle_FWFT ==
  note: We needed a FIFO which brings the valid data automatically to the output.
      | The regular XILINX Fifos are not FWFT (First Word Fall Through).
      | We tried to make one but it was really hard to make one agreeing with the exact specs.
      | This module which we have named it Trickle_FWFT Fifo works very similiarly with minor
      | differences which servers our purpose here in the DRAM VACC module.
  note: The real depth of this module is depth+1.
      | The valid signal will go high with one cycle delay.
  din : Inport
  we : Inport  Port=2
  ack : Inport  Port=3
  reset : Inport  Port=4
  Convert : xbsIndex_r4/Convert  Orientation=left  gui_display_data_type=Fixed-point  arith_type=Boolean  n_bits=8  bin_pt=6  float_type=Single  exp_bits=8  fraction_bits=24  quantization=Truncate  overflow=Wrap  en=off  latency=0  dbl_ovrd=off  pipeline=off  block_type=convert
      settings: xl_area=[0, 0, 0, 0, 0, 0, 0]  block_version=9.2.01
  Convert1 : xbsIndex_r4/Convert  gui_display_data_type=Fixed-point  arith_type=Boolean  n_bits=8  bin_pt=6  float_type=Single  exp_bits=8  fraction_bits=24  quantization=Truncate  overflow=Wrap  en=off  latency=0  dbl_ovrd=off  pipeline=off  block_type=convert
      settings: xl_area=[0, 0, 0, 0, 0, 0, 0]  block_version=9.2.01
  Convert2 : xbsIndex_r4/Convert  gui_display_data_type=Fixed-point  arith_type=Boolean  n_bits=8  bin_pt=6  float_type=Single  exp_bits=8  fraction_bits=24  quantization=Truncate  overflow=Wrap  en=off  latency=0  dbl_ovrd=off  pipeline=off  block_type=convert
      settings: xl_area=[0, 0, 0, 0, 0, 0, 0]  block_version=9.2.01
  FIFO : xbsIndex_r4/FIFO  performance_options=Standard_FIFO  depth=512  percent_nbits=1  rst=on  en=off  use_dcount=off  use_percent_full_port=on  use_almost_empty=off  almost_empty_thresh=2  use_almost_full=off  almost_full_thresh=14  dbl_ovrd=off  mem_type=Block RAM  explicit_period=on  period=1  block_type=fifo
      settings: xl_area=[0, 0, 0, 0, 0, 0, 0]  block_version=9.2.01
  Inverter3 : xbsIndex_r4/Inverter  en=off  latency=0  dbl_ovrd=off  block_type=inv
      settings: xl_area=[0, 0, 0, 0, 0, 0, 0]  block_version=9.2.01
  Logical2 : xbsIndex_r4/Logical  logical_function=OR  inputs=2  en=off  latency=0  precision=Full  arith_type=Unsigned  n_bits=8  bin_pt=2  align_bp=on  dbl_ovrd=off  block_type=logical
      settings: xl_area=[0, 0, 0, 0, 0, 0, 0]  block_version=9.2.01
  not_valid : xbsIndex_r4/Register  init=1  rst=on  en=on  dbl_ovrd=off  block_type=register
      settings: xl_area=[0, 0, 0, 0, 0, 0, 0]  block_version=9.2.01
  warn period Convert0 : xbsReplacements_r4/Warning  SystemSampleTime=-1  period=1
  warn period Logical20 : xbsReplacements_r4/Warning  SystemSampleTime=-1  period=1
  warn period not_valid0 : xbsReplacements_r4/Warning  SystemSampleTime=-1  period=1
  data_out : Outport
  valid : Outport  Port=2
  full : Outport  Port=3
  %full : Outport  Port=4
  wires:
  din/1 -> FIFO/1
  we/1 -> FIFO/2
  FIFO/2 -> not_valid/1
  ack/1 -> Convert2/1
  FIFO/1 -> data_out/1
  FIFO/4 -> full/1
  Inverter3/1 -> valid/1
  reset/1 -> FIFO/4, not_valid/2
  Logical2/1 -> FIFO/3, not_valid/3
  not_valid/1 -> Convert1/1
  Convert/1 -> Logical2/1
  FIFO/3 -> %full/1
  Convert1/1 -> Inverter3/1, Convert/1
  Convert2/1 -> Logical2/2
